simulink model "trms_model_pid_bancada"  (R2025b)
settings: Solver=ode4  StartTime=0.0  StopTime=11  FixedStep=0.001  RelTol=1e-3
values from neighbouring files (symbols this model uses):
  C_c = evalin('base', 'C_c')    [trms_equilibrium.m]    (also in trms_params.m = 0.021)
  CR_m_neg = evalin('base', 'CR_m_neg')    [trms_equilibrium.m]    (also in trms_params.m = 4.5047e-07)
  CR_m_pos = evalin('base', 'CR_m_pos')    [trms_equilibrium.m]    (also in trms_params.m = 5.0582e-07)
  CR_t_neg = 9.9176e-8    (= 9.9176e-08)    [trms_params.m]
  CR_t_pos = 9.7031e-8    (= 9.7031e-08)    [trms_params.m]
  CT_m_neg = evalin('base', 'CT_m_neg')    [trms_equilibrium.m]    (also in trms_params.m = 8.9974e-06)
  CT_m_pos = evalin('base', 'CT_m_pos')    [trms_equilibrium.m]    (also in trms_params.m = 1.4971e-05)
  CT_t_neg = 2.3046e-6    (= 2.3046e-06)    [trms_params.m]
  CT_t_pos = 3.7755e-6    (= 3.7755e-06)    [trms_params.m]
  f_cphi = 1.1758e-5    (= 1.1758e-05)    [trms_params.m]
  f_cpsi = 4.0548e-4    (= 0.00040548)    [trms_params.m]
  f_s = 3.48*f_cpsi    (= 0.0014110704)    [trms_params.m]
  f_vm = evalin('base', 'f_vm')    [trms_equilibrium.m]    (also in trms_params.m = 4.1993e-06)
  f_vphi = 2.60e-2    (= 0.026)    [trms_params.m]
  f_vpsi = 4.2150e-4    (= 0.0004215)    [trms_params.m]
  f_vt = 3.2498e-6    (= 3.2498e-06)    [trms_params.m]
  G_y = evalin('base', 'G_y')    [trms_equilibrium.m]    (also in trms_params.m = 0.15032)
  G_z = evalin('base', 'G_z')    [trms_equilibrium.m]    (also in trms_params.m = -0.25254)
  H_y = 6.6120e-3    (= 0.006612)    [trms_params.m]
  H_z = -1.5446e-3    (= -0.0015446)    [trms_params.m]
  I_c = 8.3286e-2    (= 0.083286)    [trms_params.m]
  I_m1 = 1.7249e-4    (= 0.00017249)    [trms_params.m]
  I_phi = 2.1117e-2    (= 0.021117)    [trms_params.m]
  I_psi = 6.1644e-2    (= 0.061644)    [trms_params.m]
  I_t1 = 3.2170e-5    (= 3.217e-05)    [trms_params.m]
  k_tm = evalin('base', 'k_tm')    [trms_equilibrium.m]    (also in trms_params.m = 0.0202)
  k_tt = 0.0202    [trms_params.m]
  k_um = evalin('base', 'k_um')    [trms_equilibrium.m]    (also in trms_params.m = 8.5)
  k_ut = 6.5    [trms_params.m]
  k_vm = evalin('base', 'k_vm')    [trms_equilibrium.m]    (also in trms_params.m = 0.0202)
  k_vt = 0.0202    [trms_params.m]
  Kd_pitch = 8    [trms_params.m]
  Ki_pitch = 6    [trms_params.m]
  Kp_pitch = 4    [trms_params.m]
  l_m = evalin('base', 'l_m')    [trms_equilibrium.m]    (also in trms_params.m = 0.254)
  l_t = 0.275    [trms_params.m]
  mascara = ones(6,1)    [trms_params.m]
  modo = 1    [trms_params.m]
  phi_0 = evalin('base', 'phi_0')    [confere_params.m]    (also in trms_equilibrium.m; trms_params.m = 0.03011)
  psi_0 = evalin('base', 'psi_0')    [confere_params.m]    (also in trms_params.m = -atan(G_y/abs(G_z)))
  R = evalin('base', 'R')    [trms_equilibrium.m]    (also in trms_params.m = 8)
  ref_pitch = 0.4    [trms_params.m]
  t_degrau = 10    [trms_params.m]
  v_s = 0.05    [trms_params.m]
  x0 = evalin('base', 'x0')    [confere_params.m]    (also in trms_equilibrium.m = [psi_eq; phi_eq; om_m_eq; 0; 0; 0]; trms_params.m = [psi_0; phi_0; 0; 0; 0; 0])
undefined symbols (not defined in the file or in its folder): DiscIntNeverNeededParam, dspblkCoreblockFVToolHelper, gcbh
libraries: simulink x1
settings Model: Creator=clara.marigo  LastModifiedBy=tmcla

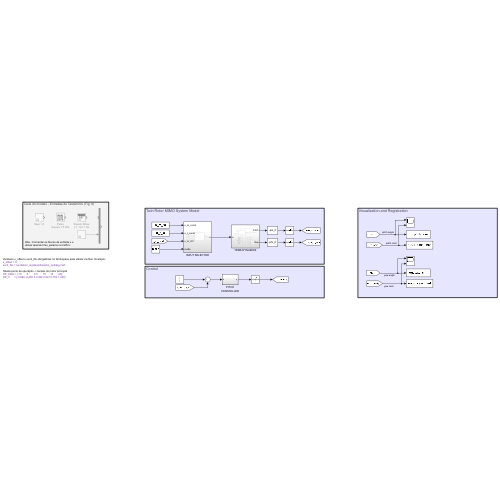
[thumbnail: Simulink's stored preview of the top-level diagram]
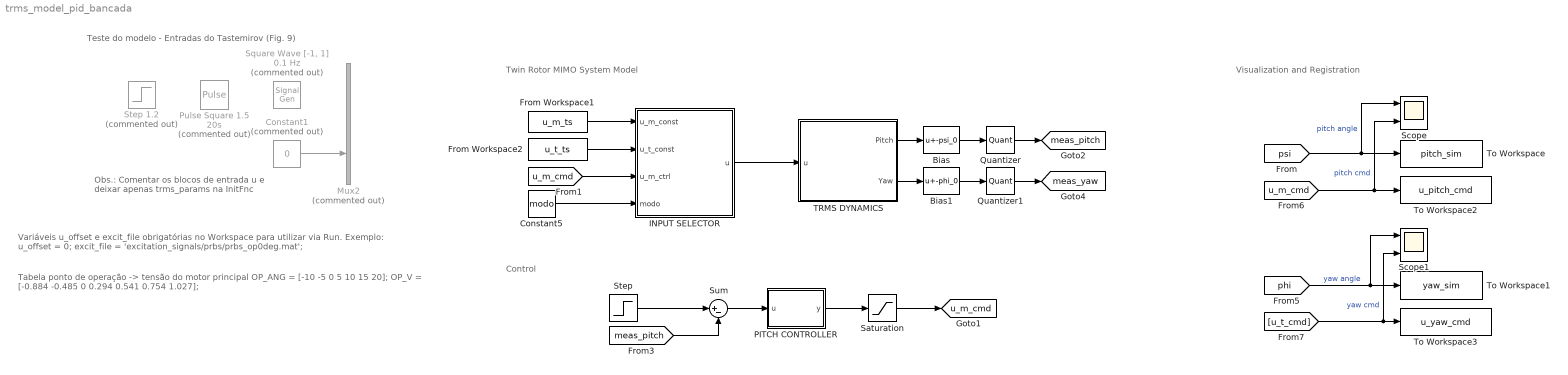
== system trms_model_pid_bancada ==
  note: Tabela ponto de operação -> tensão do motor principal
      | OP_ANG = [-10 -5 0 5 10 15 20];
      | OP_V = [-0.884 -0.485 0 0.294 0.541 0.754 1.027];
  note: Variáveis u_offset e excit_file obrigatórias no Workspace para utilizar via Run. Exemplo:
      | u_offset = 0;
      | excit_file = 'excitation_signals/prbs/prbs_op0deg.mat';
  note: Obs.: Comentar os blocos de entrada u e deixar apenas trms_params na InitFnc
  note: Twin Rotor MIMO System Model
  note: Teste do modelo - Entradas do Tastemirov (Fig. 9)
  note: Control
  note: Visualization and Registration
  Bias : Bias  Bias=-psi_0  SaturateOnIntegerOverflow=off
  Bias1 : Bias  Bias=-phi_0  SaturateOnIntegerOverflow=off
  Constant1 : Constant  Commented=on  Value=0
  Constant5 : Constant  Value=modo
  From Workspace1 : FromWorkspace  VariableName=u_m_ts  Interpolate=off  OutputAfterFinalValue=Holding final value
  From Workspace2 : FromWorkspace  VariableName=u_t_ts  Interpolate=off  OutputAfterFinalValue=Holding final value
  INPUT SELECTOR : Subsystem
  Mux2 : Mux  Commented=on  Inputs=2
  PITCH CONTROLLER : Subsystem
  Pulse Square 1.5 20s : DiscretePulseGenerator  Commented=on  PulseType=Time based  Amplitude=1.5  Period=100  PulseWidth=20
  Quantizer : Quantizer  QuantizationInterval=2*pi/2048
  Quantizer1 : Quantizer  QuantizationInterval=2*pi/2048
  Saturation : Saturate  UpperLimit=2.5  LowerLimit=-2.5
  Scope : Scope  NumInputPorts=2
      settings: ActiveDisplayYMinimum=-0.748007571257962  ActiveDisplayYMaximum=0.08311195236199577
  Scope1 : Scope  NumInputPorts=2
      settings: ActiveDisplayYMinimum=-1.1544179589662236  ActiveDisplayYMaximum=0.38839915128191682
  "Square Wave [-1, 1] 0.1 Hz" : SignalGenerator  Commented=on  WaveForm=square  Frequency=0.1  VectorParams1D=off
  Step : Step  Time=t_degrau  After=ref_pitch  SampleTime=0.001
  Step 1.2 : Step  Commented=on  Time=0  Before=-0.54  After=1.25  SampleTime=0.1
  Sum : Sum  Inputs=|+-
  TRMS DYNAMICS : Subsystem
  To Workspace : ToWorkspace  VariableName=pitch_sim  SaveFormat=Timeseries  SampleTime=-1
  To Workspace1 : ToWorkspace  VariableName=yaw_sim  SaveFormat=Timeseries  SampleTime=-1
  To Workspace2 : ToWorkspace  VariableName=u_pitch_cmd  SaveFormat=Timeseries  SampleTime=-1
  To Workspace3 : ToWorkspace  VariableName=u_yaw_cmd  SaveFormat=Timeseries  SampleTime=-1
  tag scope: meas_pitch=global, meas_yaw=global, u_m_cmd=global
  wires:
  [psi] -> To Workspace/1, Scope/1  "pitch angle"
  Constant1/1 -> Mux2/2
  [meas_pitch] -> Sum/2
  [phi] -> Scope1/1, To Workspace1/1  "yaw angle"
  [u_m_cmd] -> Scope/2, To Workspace2/1  "pitch cmd"
  [u_t_cmd] -> Scope1/2, To Workspace3/1  "yaw cmd"
  Step/1 -> Sum/1
  Bias/1 -> Quantizer/1
  TRMS DYNAMICS/1(Pitch) -> Bias/1
  Sum/1 -> PITCH CONTROLLER/1(u)
  PITCH CONTROLLER/1(y) -> Saturation/1
  Quantizer/1 -> [meas_pitch]
  Saturation/1 -> [u_m_cmd]
  Quantizer1/1 -> [meas_yaw]
  TRMS DYNAMICS/2(Yaw) -> Bias1/1
  Bias1/1 -> Quantizer1/1
  INPUT SELECTOR/1(u) -> TRMS DYNAMICS/1(u)
  From Workspace1/1 -> INPUT SELECTOR/1(u_m_const)
  From Workspace2/1 -> INPUT SELECTOR/2(u_t_const)
  [u_m_cmd] -> INPUT SELECTOR/3(u_m_ctrl)
  Constant5/1 -> INPUT SELECTOR/4(modo)

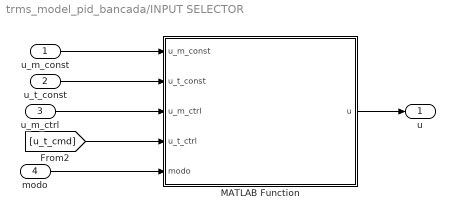
== system trms_model_pid_bancada/INPUT SELECTOR ==
  u_m_const : Inport
  u_t_const : Inport  Port=2
  u_m_ctrl : Inport  Port=3
  modo : Inport  Port=4
  MATLAB Function : MATLAB Function  TreatAsAtomicUnit=on
  u : Outport
  wires:
  [u_t_cmd] -> MATLAB Function/4(u_t_ctrl)
  u_m_const/1 -> MATLAB Function/1(u_m_const)
  modo/1 -> MATLAB Function/5(modo)
  u_m_ctrl/1 -> MATLAB Function/3(u_m_ctrl)
  u_t_const/1 -> MATLAB Function/2(u_t_const)
  MATLAB Function/1(u) -> u/1

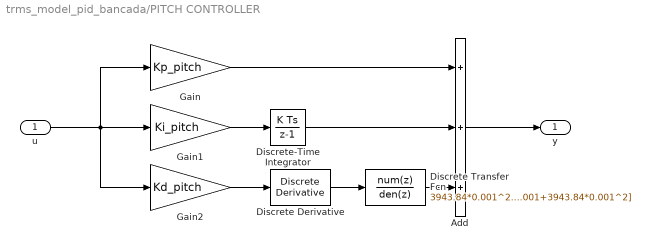
== system trms_model_pid_bancada/PITCH CONTROLLER ==
  u : Inport
  Add : Sum  Inputs=+++
  Discrete Transfer Fcn : DiscreteTransferFcn  LoadFcn=dspblkCoreblockFVToolHelper(gcbh,'load');  Numerator=3943.84*0.001^2  Denominator=[1, -2+44.4*0.001, 1-44.4*0.001+3943.84*0.001^2]
      settings: CopyFcn=dspblkCoreblockFVToolHelper(gcbh,'copy');  DeleteFcn=dspblkCoreblockFVToolHelper(gcbh,'close');  ModelCloseFcn=dspblkCoreblockFVToolHelper(gcbh,'close');  PreSaveFcn=dspblkCoreblockFVToolHelper(gcbh,'presave');  PostSaveFcn=dspblkCoreblockFVToolHelper(gcbh,'postsave');  CloseFcn=dspblkCoreblockFVToolHelper(gcbh,'close');
  Discrete Derivative : simulink/Discrete/Discrete Derivative  gainval=1.0  ICPrevScaledInput=0.0  OutMin=[]  OutMax=[]  OutDataType=fixdt(1, 16)  OutScaling=2^-10  DoSatur=off
  Discrete-Time Integrator : DiscreteIntegrator  SampleTime=0.001  ICPrevOutput=DiscIntNeverNeededParam  ICPrevScaledInput=DiscIntNeverNeededParam
  Gain : Gain  Gain=Kp_pitch
  Gain1 : Gain  Gain=Ki_pitch
  Gain2 : Gain  Gain=Kd_pitch
  y : Outport
  wires:
  Add/1 -> y/1
  u/1 -> Gain/1, Gain2/1, Gain1/1
  Gain1/1 -> Discrete-Time Integrator/1
  Discrete-Time Integrator/1 -> Add/2
  Gain2/1 -> Discrete Derivative/1
  Discrete Transfer Fcn/1 -> Add/3
  Discrete Derivative/1 -> Discrete Transfer Fcn/1
  Gain/1 -> Add/1

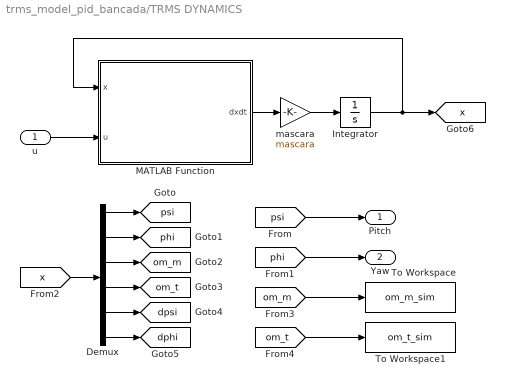
== system trms_model_pid_bancada/TRMS DYNAMICS ==
  u : Inport
  Demux : Demux  Outputs=6
  Integrator : Integrator  InitialCondition=x0
  MATLAB Function : MATLAB Function  TreatAsAtomicUnit=on
  To Workspace : ToWorkspace  VariableName=om_m_sim  SaveFormat=Timeseries  SampleTime=-1
  To Workspace1 : ToWorkspace  VariableName=om_t_sim  SaveFormat=Timeseries  SampleTime=-1
  mascara : Gain  Gain=mascara
  Pitch : Outport
  Yaw : Outport  Port=2
  tag scope: dphi=global, dpsi=global, om_m=global, om_t=global, phi=global, psi=global, x=global
  wires:
  [x] -> Demux/1
  Demux/2 -> [phi]
  Demux/1 -> [psi]
  Demux/3 -> [om_m]
  Demux/5 -> [dpsi]
  Demux/6 -> [dphi]
  Demux/4 -> [om_t]
  u/1 -> MATLAB Function/2(u)
  [phi] -> Yaw/1
  [psi] -> Pitch/1
  mascara/1 -> Integrator/1
  Integrator/1 -> [x], MATLAB Function/1(x)
  MATLAB Function/1(dxdt) -> mascara/1
  [om_m] -> To Workspace/1
  [om_t] -> To Workspace1/1

== matlab function trms_model_pid_bancada/INPUT SELECTOR/MATLAB Function ==
  data: u_m_const input; u output; u_t_const input; u_m_ctrl input; u_t_ctrl input; modo input
function u = trms_sel_entrada(u_m_const, u_t_const, u_m_ctrl, u_t_ctrl, modo)
% TRMS_SEL_ENTRADA Seleciona a origem do comando de cada eixo do TRMS.
%
% Entradas (escalares):
%   u_m_const - comando de malha aberta do rotor principal [V]
%   u_t_const - comando de malha aberta do rotor de cauda  [V]
%   u_m_ctrl  - saida do controlador de pitch              [V]
%   u_t_ctrl  - saida do controlador de yaw                [V]
%   modo      - seletor de configuracao da malha:
%               0 = pitch malha aberta,  yaw malha aberta
%               1 = pitch malha fechada, yaw malha aberta
%               2 = pitch malha aberta,  yaw malha fechada
%               3 = pitch malha fechada, yaw malha fechada
%
% Saida:
%   u - vetor 2x1 [u_m; u_t] entregue ao bloco da planta
%
% Valor de modo nao reconhecido resulta em malha aberta nos dois eixos,
% que e a condicao segura (nenhuma realimentacao ativa).

u_m = u_m_const;
u_t = u_t_const;

if modo == 1
    u_m = u_m_ctrl;
elseif modo == 2
    u_t = u_t_ctrl;
elseif modo == 3
    u_m = u_m_ctrl;
    u_t = u_t_ctrl;
end

u = [u_m; u_t];

== matlab function trms_model_pid_bancada/TRMS DYNAMICS/MATLAB Function ==
  data: x input size=6; u input; dxdt output size=6; I_m1 parameter; I_t1 parameter; I_psi parameter; I_phi parameter; I_c parameter; G_z parameter; G_y parameter; H_z parameter; H_y parameter; f_vpsi parameter; f_cpsi parameter; f_vphi parameter; f_cphi parameter; f_vm parameter; f_vt parameter; CT_m_pos parameter; CT_m_neg parameter; CT_t_pos parameter; CT_t_neg parameter; CR_m_pos parameter; CR_m_neg parameter; CR_t_pos parameter; CR_t_neg parameter; C_c parameter; phi_0 parameter; R parameter; k_vm parameter; k_vt parameter; k_tm parameter; k_tt parameter; k_um parameter; k_ut parameter; l_m parameter; l_t parameter; f_s parameter; v_s parameter
function dxdt = trms_dynamics(x, u, ...
    I_m1, I_t1, I_psi, I_phi, I_c, ...
    G_z, G_y, H_z, H_y, ...
    f_vpsi, f_cpsi, f_vphi, f_cphi, f_vm, f_vt, ...
    CT_m_pos, CT_m_neg, CT_t_pos, CT_t_neg, ...
    CR_m_pos, CR_m_neg, CR_t_pos, CR_t_neg, ...
    C_c, phi_0, ...
    R, k_vm, k_vt, k_tm, k_tt, k_um, k_ut, l_m, l_t, f_s, v_s)

%% 1. Extração dos estados 

psi   = x(1);   % ângulo de pitch            [rad]
phi   = x(2);   % ângulo de yaw              [rad]
om_m  = x(3);   % velocidade do main rotor   [rad/s]
om_t  = x(4);   % velocidade do tail rotor   [rad/s]
dpsi  = x(5);   % velocidade angular de pitch [rad/s]
dphi  = x(6);   % velocidade angular de yaw  [rad/s]

dxdt = zeros(6, 1);

%% 2. Tensões e correntes dos motores (eq. 3) 

v_m = k_um * u(1);              % tensão aplicada ao main rotor [V]
i_m = (v_m - k_vm * om_m) / R;  % corrente da armadura, main rotor [A]

v_t = k_ut * u(2);              % tensao aplicada ao tail rotor [V]
i_t = (v_t - k_vt * om_t) / R;  % corrente da armadura, tail rotor [A]

%% 3. Coeficientes aerodinâmicos dependentes do sinal
%   Os coeficientes de empuxo (CT) e torque de reação (CR) são assimétricos,
%   as hélices produzem forças diferentes dependendo da direção de rotação.

if om_m >= 0
    CT_m = CT_m_pos;
    CR_m = CR_m_pos;
else
    CT_m = CT_m_neg;
    CR_m = CR_m_neg;
end

if om_t >= 0
    CT_t = CT_t_pos;
    CR_t = CR_t_pos;
else
    CT_t = CT_t_neg;
    CR_t = CR_t_neg;
end

%% 3b. Atrito de pitch: Coulomb + estatico (aproximacao suave)
%   Modelo estatico geral do survey de atritos (Iurian et al., 2005), na
%   forma continua tipo Stribeck. Perto de dpsi=0 o atrito sobe ate o nivel
%   estatico f_s (maior que o cinetico f_cpsi); conforme |dpsi| cresce, o
%   acrescimo estatico decai exponencialmente e sobra so o Coulomb f_cpsi.
%   v_s (velocidade de Stribeck) controla a largura dessa transicao.
%   Com f_s = f_cpsi, o termo estatico zera e recai no modelo Coulomb puro
%   (util como teste de sanidade contra o modelo antigo).
atrito_coulomb_estatico = (f_cpsi + (f_s - f_cpsi) * exp(-abs(dpsi)/v_s)) * sign(dpsi);

%% 4. Matriz de inércia (eqs. 28-31) 
%   Incógnitas: [ddpsi; ddphi; dom_m; dom_t]

coupling = H_z * cos(psi) + H_y * sin(psi);   % Coupling das eqs. (28-29)

M = [ I_psi,      -coupling,               0,             I_t1; ...
      -coupling,  I_phi + I_c*cos(psi)^2,  I_m1*cos(psi), 0;   ...
       0,         I_m1*cos(psi),           I_m1,          0;   ...
       I_t1,      0,                       0,             I_t1 ];

%% 5. Vetores do lado direito das equações (eqs. 28-31) ───────────────────

% Pitch (eq. 28)
RHS_psi = ...
    - (1/2) * I_c * dphi^2 * sin(2*psi) ...    % centrifugo/Coriolis
    - I_m1 * om_m * dphi * sin(psi) ...        % giroscopico (main rotor)
    + G_z * sin(psi) ...                       % torque gravitacional
    - G_y * cos(psi) ...                       % torque gravitacional
    + CT_m * om_m * abs(om_m) * l_m ...        % empuxo do main rotor
    - CR_t * om_t * abs(om_t) ...              % reacao do tail rotor no pitch
    - f_vpsi * dpsi ...                        % atrito viscoso
    - atrito_coulomb_estatico;                 % atrito Coulomb + estatico (suave)

% Yaw (eq. 29)
RHS_phi = ...
    - (H_z * sin(psi) - H_y * cos(psi)) * dpsi^2 ... % centrifugo (viga pivotante)
    + I_c * dphi * dpsi * sin(2*psi) ...             % Coriolis
    + I_m1 * om_m * dpsi * sin(psi) ...              % giroscopico (main rotor)
    + CT_t * om_t * abs(om_t) * l_t * cos(psi) ...   % empuxo do tail rotor
    - CR_m * om_m * abs(om_m) * cos(psi) ...         % reacao do main rotor no yaw
    - f_vphi * dphi ...                              % atrito viscoso
    - f_cphi * sign(dphi) ...                        % atrito de Coulomb
    - C_c * (phi - phi_0);                           % torque do cabo

% Main rotor (eq. 30)
RHS_30 = I_m1 * dphi * dpsi * sin(psi) ...    % Coriolis 
       + k_tm * i_m ...                       % torque eletromecânico
       - f_vm * om_m ...                      % atrito viscoso
       - CR_m * om_m * abs(om_m);             % arrasto aerodinâmico

% Tail rotor (eq. 31)
RHS_31 = k_tt * i_t ...                       % torque eletromecânico
       - f_vt * om_t ...                      % atrito viscoso
       - CR_t * om_t * abs(om_t);             % arrasto aerodinâmico

%% 6. Resolução do sistema 
% Equivalente à inversão da matriz de inércia variante no tempo

sol   = M \ [RHS_psi; RHS_phi; RHS_30; RHS_31];
ddpsi = sol(1);
ddphi = sol(2);
dom_m = sol(3);
dom_t = sol(4);

%% 7. Montagem do vetor dxdt ──────────────────────────────────────────────

dxdt(1) = dpsi;   % (igual a x(5))
dxdt(2) = dphi;   % (igual a x(6))
dxdt(3) = dom_m;  % aceleração angular do main rotor  [rad/s^2]
dxdt(4) = dom_t;  % aceleração angular do tail rotor  [rad/s^2]
dxdt(5) = ddpsi;  % aceleração angular de pitch       [rad/s^2]
dxdt(6) = ddphi;  % aceleração angular de yaw         [rad/s^2]


end
